simulink model "ESSSimulation_NCR"  (R2025a)
settings: Solver=VariableStepAuto  StartTime=0.0  StopTime=1800  RelTol=1e-3
undefined symbols (not defined in the file or in its folder): battery_builder_rtmsupport, gcbh
libraries: NCR18650BD_98S45P_Library_lib x14, fl_lib x4, nesl_utility x4, simulink x1, SignalEditorBlockLib x1
(part 1 of 2)
settings Model: Creator=saarv  LastModifiedBy=saarv

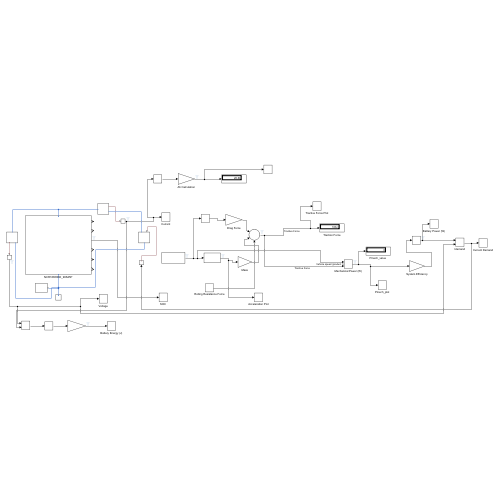
[thumbnail: Simulink's stored preview of the top-level diagram]
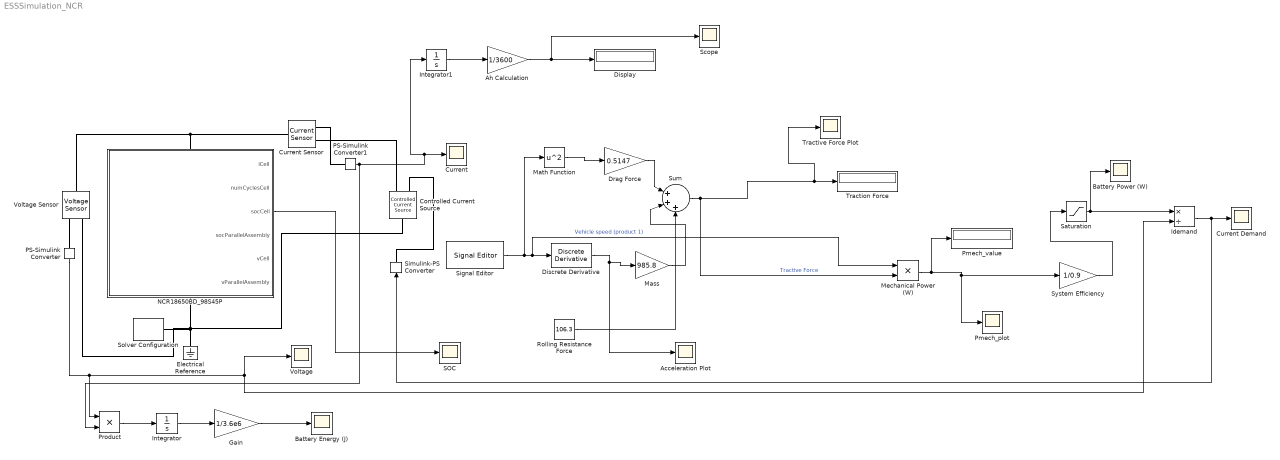
== system ESSSimulation_NCR ==
  Acceleration Plot : Scope
      settings: ActiveDisplayYMinimum=-1  ActiveDisplayYMaximum=1  DataLoggingVariableName=ScopeData3
  Ah Calculation : Gain  Gain=1/3600
  Battery Energy (J) : Scope
      settings: ActiveDisplayYMinimum=-1  ActiveDisplayYMaximum=1  DataLoggingVariableName=ScopeData8
  Battery Power (W) : Scope
      settings: ActiveDisplayYMinimum=-1660.4480803591648  ActiveDisplayYMaximum=14944.032723232487  DataLoggingVariableName=ScopeData6
  Controlled Current Source : fl_lib/Electrical/Electrical Sources/Controlled Current Source
  Current : Scope
      settings: ActiveDisplayYMinimum=-4.1863215438734489  ActiveDisplayYMaximum=37.676893894861045
  Current Demand : Scope
      settings: ActiveDisplayYMinimum=-4.1462072619256087  ActiveDisplayYMaximum=37.315865357330487  DataLoggingVariableName=ScopeData7
  Current Sensor : fl_lib/Electrical/Electrical Sensors/Current Sensor
  Discrete Derivative : simulink/Discrete/Discrete Derivative  gainval=1.0  ICPrevScaledInput=0.0  OutMin=[]  OutMax=[]  OutDataType=fixdt(1, 16)  OutScaling=2^-10  DoSatur=off
  Display : Display
  Drag Force : Gain  Gain=0.5147
  Electrical Reference : fl_lib/Electrical/Electrical Elements/Electrical Reference
  Gain : Gain  Gain=1/3.6e6
  Idemand : Product  Inputs=*/
  Integrator : Integrator
  Integrator1 : Integrator
  Mass : Gain  Gain=985.8
  Math Function : Math  Operator=square
  Mechanical Power (W) : Product
  NCR18650BD_98S45P : Subsystem  LoadFcn=battery_builder_rtmsupport('loadfcn',gcbh);
      settings: CopyFcn=battery_builder_rtmsupport('copyfcn',gcbh);  PreCopyFcn=battery_builder_rtmsupport('precopyfcn',gcbh);  PreDeleteFcn=battery_builder_rtmsupport('predeletefcn',gcbh);  PortSchema="{\"entries\":[{\"content\":{\"sides\":[{\"content\":{\"connectorIds\":[\"LConn1\"]},\"type\":\"ConnectorPlacement.EquallySpacedRectSide\",\"uuid\":\"9e7041d5-d3d9-4996-bd95-b169094aaa75\"},{\"content\":{\"connectorIds\":[\"RConn1\"],\"side\":\"RIGHT\"},\"type\":\"ConnectorPlacement.EquallySpacedRectSide\",\"uuid\":\"1a9d726b-e110-445d-9094-f9af8985733a\"},{\"content\":{\"side\":\"TOP\"},\"type\":\"ConnectorPlacement.EquallySpacedRectSide\",\"uuid\":\"c9094138-05f6-46bf-9d7c-2f9307e18b10\"},{\"content\":{\"connectorIds\":[\"Out1\",\"Out2\",\"Out3\",\"Out4\",\"Out5\",\"Out6\"],\"side\":\"BOTTOM\"},\"type\":\"ConnectorPlacement.EquallySpacedRectSide\",\"uuid\":\"12959d5d-2702-4b18-986c-5ba3b231edc9\"}]},\"type\":\"ConnectorPlacement.EquallySpacedConnector\",\"uuid\":\"b4792a63-91de-4aa8-9329-1ac229a09e41\"}],\"packageUris\":[\"http://schema.mathworks.com/mf0/Connector/R2020b\"],\"version\":\"1.0\"}"
      mask Display: image('$imagefile')
  PS-Simulink Converter : nesl_utility/PS-Simulink Converter  PhysicalDomain=network_engine_domain  SubClassName=ps_output  LeftPortType=input  RightPortType=output  PseudoPeriodic=off  Frequencies=[]  VectorFormat=inherit  Unit=inherit  AffineConversion=off
  PS-Simulink Converter1 : nesl_utility/PS-Simulink Converter  PhysicalDomain=network_engine_domain  SubClassName=ps_output  LeftPortType=input  RightPortType=output  PseudoPeriodic=off  Frequencies=[]  VectorFormat=inherit  Unit=inherit  AffineConversion=off
  Pmech_plot : Scope
      settings: ActiveDisplayYMinimum=-4360.824190842518  ActiveDisplayYMaximum=13768.120664078046  DataLoggingVariableName=ScopeData5
  "Pmech_value " : Display
  Product : Product
  Rolling Resistance Force : Constant  Value=106.3
  SOC : Scope
      settings: ActiveDisplayYMinimum=0.95619971788129954  ActiveDisplayYMaximum=1.0048666980131891  DataLoggingVariableName=ScopeData2
  Saturation : Saturate  UpperLimit=inf  LowerLimit=0
  Scope : Scope
      settings: ActiveDisplayYMinimum=-1  ActiveDisplayYMaximum=1  DataLoggingVariableName=ScopeData9
  Signal Editor : SignalEditorBlockLib/Signal Editor  FileName=EV_DriveProfiles.mat  ActiveScenario=SportProfile  ActiveSignal=VehicleSpeed  IsBus=off  OutputBusObjectStr=Bus: BusObject  SampleTime=10  ZeroCross=off  OutputAfterFinalValue=Setting to zero  Unit=m/s  PreserveSignalName=on  ApplySigPropsToAllScenarios=on  ApplySigPropsToAllSignals=off  SignalPropertySource=Dialog parameters
  Simulink-PS Converter : nesl_utility/Simulink-PS Converter  PhysicalDomain=network_engine_domain  SubClassName=ps_input  LeftPortType=input  RightPortType=output  PseudoPeriodic=off  Frequencies=[]  NoiseDistribution=none  NoiseParameters=[]  Unit=A  AffineConversion=off  FilteringAndDerivatives=provide  SimscapeFilterOrder=1  InputFilterTimeConstant=0.001  UdotUserProvided=0
  Solver Configuration : nesl_utility/Solver Configuration  PhysicalDomain=network_engine_domain  SubClassName=solver  LeftPortType=input  RightPortType=generic  Tones=[]  Harmonics=[]  SimulateNoise=off  Profile=off  UseLocalSampling=off  EnableSwitchedLinearOptims=on  FrequencyDomain=off  UseCCode=off  RelTol=0.001  AbsTol=0.001  MinStep=1e-09  ToWorkspace=off  RevertToSquareIcSolve=off  NumHomotopyIterations=100  PhasorMode=off  PhasorModeNumHarmonics=1  ConsistencySolver=NEWTON_XTOL_AFTER_FTOL  IndexReductionMethod=DerivativeReplacement  DoDC=off  ResidualTolerance=1e-09  ConsistencyTolSource=GLOBAL  ConsistencyAbsTol=0.001  ConsistencyRelTol=0.001  ConsistencyTolFactor=0.001  UseLocalSolver=off  LocalSolverChoice=NE_BACKWARD_EULER_ADVANCER  ResolveIndetEquations=on  FunctionEvalNumThread=1  LocalSolverSampleTime=0.001  DoFixedCost=off  MaxNonlinIter=3  MaxModeIter=2  ComputeImpulses=off  ImpulseIterations=2  LinearAlgebra=auto  LinearAlgebraNumThread=0  EquationFormulation=NE_TIME_EF  DelaysMemoryBudget=1024  AutomaticFiltering=on  FilteringTimeConstant=0.001  PartitionStorageMethod=AS_NEEDED  PartitionMemoryBudget=1024  PartitionMethod=ROBUST  MultibodyUseLocalSolver=off  MultibodyLocalSolverChoice=ODE1  MultibodyLocalSolverSampleTime=0.001
  Sum : Sum  Inputs=|+++
  System Efficiency : Gain  Gain=1/0.9
  Traction Force : Display
  Tractive Force Plot : Scope
      settings: ActiveDisplayYMinimum=-1  ActiveDisplayYMaximum=1  DataLoggingVariableName=ScopeData4
  Voltage : Scope
      settings: ActiveDisplayYMinimum=395.47317775463534  ActiveDisplayYMaximum=402.99624691615156
  Voltage Sensor : fl_lib/Electrical/Electrical Sensors/Voltage Sensor
  wires:
  PS-Simulink Converter/1 -> Product/1, Idemand/2, Voltage/1
  PS-Simulink Converter1/1 -> Product/2, Integrator1/1, Current/1
  Signal Editor/1 -> Math Function/1, Discrete Derivative/1, Mechanical Power (W)/1  "Vehicle speed (product 1)"
  Math Function/1 -> Drag Force/1
  Discrete Derivative/1 -> Acceleration Plot/1, Mass/1
  Drag Force/1 -> Sum/1
  Mass/1 -> Sum/2
  Rolling Resistance Force/1 -> Sum/3
  Sum/1 -> Mechanical Power (W)/2, Tractive Force Plot/1, Traction Force/1  "Tractive Force"
  Mechanical Power (W)/1 -> System Efficiency/1, Pmech_plot/1, "Pmech_value "/1
  System Efficiency/1 -> Saturation/1
  Saturation/1 -> Idemand/1, Battery Power (W)/1
  Idemand/1 -> Simulink-PS Converter/1, Current Demand/1
  Product/1 -> Integrator/1
  Integrator/1 -> Gain/1
  Gain/1 -> Battery Energy (J)/1
  Integrator1/1 -> Ah Calculation/1
  Ah Calculation/1 -> Scope/1, Display/1
  NCR18650BD_98S45P/3(socCell) -> SOC/1
  connections:
  Voltage Sensor/LConn1 -- NCR18650BD_98S45P/LConn1 -- Current Sensor/LConn1
  Electrical Reference/LConn1 -- NCR18650BD_98S45P/RConn1 -- Controlled Current Source/LConn1 -- Voltage Sensor/RConn2 -- Solver Configuration/RConn1
  Simulink-PS Converter/RConn1 -- Controlled Current Source/RConn1
  Voltage Sensor/RConn1 -- PS-Simulink Converter/LConn1
  Current Sensor/RConn1 -- PS-Simulink Converter1/LConn1
  Controlled Current Source/RConn2 -- Current Sensor/RConn2

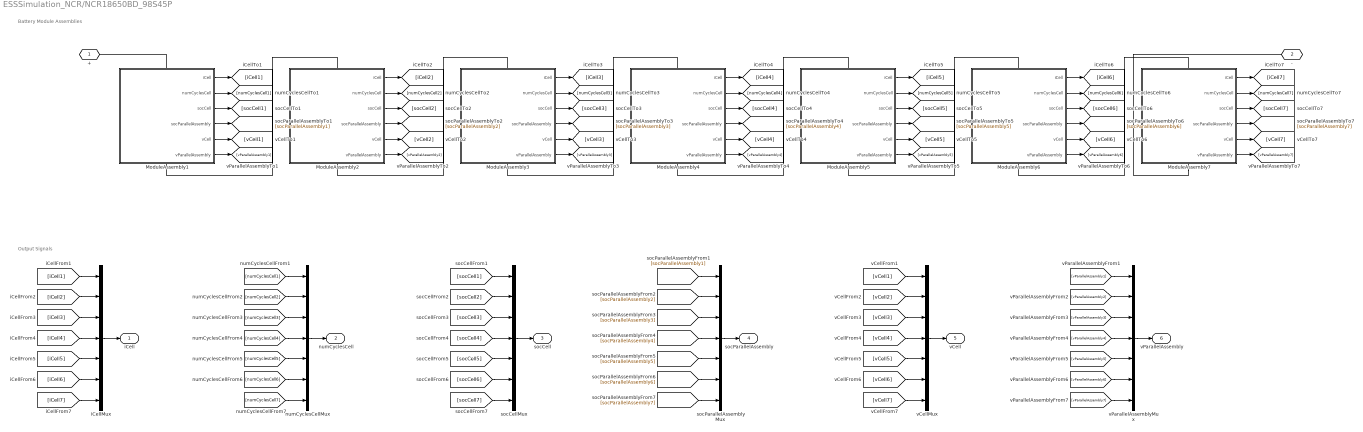
== system ESSSimulation_NCR/NCR18650BD_98S45P ==
  note: Output Signals
  note: Battery Module Assemblies
  ModuleAssembly1 : Subsystem  LoadFcn=battery_builder_rtmsupport('loadfcn',gcbh);
      settings: CopyFcn=battery_builder_rtmsupport('copyfcn',gcbh);  PreCopyFcn=battery_builder_rtmsupport('precopyfcn',gcbh);  PreDeleteFcn=battery_builder_rtmsupport('predeletefcn',gcbh);  PortSchema="{\"entries\":[{\"content\":{\"sides\":[{\"content\":{\"connectorIds\":[\"LConn1\"]},\"type\":\"ConnectorPlacement.EquallySpacedRectSide\",\"uuid\":\"9e7041d5-d3d9-4996-bd95-b169094aaa75\"},{\"content\":{\"connectorIds\":[\"RConn1\"],\"side\":\"RIGHT\"},\"type\":\"ConnectorPlacement.EquallySpacedRectSide\",\"uuid\":\"1a9d726b-e110-445d-9094-f9af8985733a\"},{\"content\":{\"side\":\"TOP\"},\"type\":\"ConnectorPlacement.EquallySpacedRectSide\",\"uuid\":\"c9094138-05f6-46bf-9d7c-2f9307e18b10\"},{\"content\":{\"connectorIds\":[\"Out1\",\"Out2\",\"Out3\",\"Out4\",\"Out5\",\"Out6\"],\"side\":\"BOTTOM\"},\"type\":\"ConnectorPlacement.EquallySpacedRectSide\",\"uuid\":\"a73cbc57-fefd-438e-a02a-7299c4782ae8\"}]},\"type\":\"ConnectorPlacement.EquallySpacedConnector\",\"uuid\":\"b4792a63-91de-4aa8-9329-1ac229a09e41\"}],\"packageUris\":[\"http://schema.mathworks.com/mf0/Connector/R2020b\"],\"version\":\"1.0\"}"
      mask Display: image('$imagefile')
  ModuleAssembly2 : Subsystem  LoadFcn=battery_builder_rtmsupport('loadfcn',gcbh);
      settings: CopyFcn=battery_builder_rtmsupport('copyfcn',gcbh);  PreCopyFcn=battery_builder_rtmsupport('precopyfcn',gcbh);  PreDeleteFcn=battery_builder_rtmsupport('predeletefcn',gcbh);  PortSchema="{\"entries\":[{\"content\":{\"sides\":[{\"content\":{\"connectorIds\":[\"LConn1\"]},\"type\":\"ConnectorPlacement.EquallySpacedRectSide\",\"uuid\":\"9e7041d5-d3d9-4996-bd95-b169094aaa75\"},{\"content\":{\"connectorIds\":[\"RConn1\"],\"side\":\"RIGHT\"},\"type\":\"ConnectorPlacement.EquallySpacedRectSide\",\"uuid\":\"1a9d726b-e110-445d-9094-f9af8985733a\"},{\"content\":{\"side\":\"TOP\"},\"type\":\"ConnectorPlacement.EquallySpacedRectSide\",\"uuid\":\"c9094138-05f6-46bf-9d7c-2f9307e18b10\"},{\"content\":{\"connectorIds\":[\"Out1\",\"Out2\",\"Out3\",\"Out4\",\"Out5\",\"Out6\"],\"side\":\"BOTTOM\"},\"type\":\"ConnectorPlacement.EquallySpacedRectSide\",\"uuid\":\"a73cbc57-fefd-438e-a02a-7299c4782ae8\"}]},\"type\":\"ConnectorPlacement.EquallySpacedConnector\",\"uuid\":\"b4792a63-91de-4aa8-9329-1ac229a09e41\"}],\"packageUris\":[\"http://schema.mathworks.com/mf0/Connector/R2020b\"],\"version\":\"1.0\"}"
      mask Display: image('moduleAssembly_1.JPG');
  ModuleAssembly3 : Subsystem  LoadFcn=battery_builder_rtmsupport('loadfcn',gcbh);
      settings: CopyFcn=battery_builder_rtmsupport('copyfcn',gcbh);  PreCopyFcn=battery_builder_rtmsupport('precopyfcn',gcbh);  PreDeleteFcn=battery_builder_rtmsupport('predeletefcn',gcbh);  PortSchema="{\"entries\":[{\"content\":{\"sides\":[{\"content\":{\"connectorIds\":[\"LConn1\"]},\"type\":\"ConnectorPlacement.EquallySpacedRectSide\",\"uuid\":\"9e7041d5-d3d9-4996-bd95-b169094aaa75\"},{\"content\":{\"connectorIds\":[\"RConn1\"],\"side\":\"RIGHT\"},\"type\":\"ConnectorPlacement.EquallySpacedRectSide\",\"uuid\":\"1a9d726b-e110-445d-9094-f9af8985733a\"},{\"content\":{\"side\":\"TOP\"},\"type\":\"ConnectorPlacement.EquallySpacedRectSide\",\"uuid\":\"c9094138-05f6-46bf-9d7c-2f9307e18b10\"},{\"content\":{\"connectorIds\":[\"Out1\",\"Out2\",\"Out3\",\"Out4\",\"Out5\",\"Out6\"],\"side\":\"BOTTOM\"},\"type\":\"ConnectorPlacement.EquallySpacedRectSide\",\"uuid\":\"a73cbc57-fefd-438e-a02a-7299c4782ae8\"}]},\"type\":\"ConnectorPlacement.EquallySpacedConnector\",\"uuid\":\"b4792a63-91de-4aa8-9329-1ac229a09e41\"}],\"packageUris\":[\"http://schema.mathworks.com/mf0/Connector/R2020b\"],\"version\":\"1.0\"}"
      mask Display: image('moduleAssembly_2.JPG');
  ModuleAssembly4 : Subsystem  LoadFcn=battery_builder_rtmsupport('loadfcn',gcbh);
      settings: CopyFcn=battery_builder_rtmsupport('copyfcn',gcbh);  PreCopyFcn=battery_builder_rtmsupport('precopyfcn',gcbh);  PreDeleteFcn=battery_builder_rtmsupport('predeletefcn',gcbh);  PortSchema="{\"entries\":[{\"content\":{\"sides\":[{\"content\":{\"connectorIds\":[\"LConn1\"]},\"type\":\"ConnectorPlacement.EquallySpacedRectSide\",\"uuid\":\"9e7041d5-d3d9-4996-bd95-b169094aaa75\"},{\"content\":{\"connectorIds\":[\"RConn1\"],\"side\":\"RIGHT\"},\"type\":\"ConnectorPlacement.EquallySpacedRectSide\",\"uuid\":\"1a9d726b-e110-445d-9094-f9af8985733a\"},{\"content\":{\"side\":\"TOP\"},\"type\":\"ConnectorPlacement.EquallySpacedRectSide\",\"uuid\":\"c9094138-05f6-46bf-9d7c-2f9307e18b10\"},{\"content\":{\"connectorIds\":[\"Out1\",\"Out2\",\"Out3\",\"Out4\",\"Out5\",\"Out6\"],\"side\":\"BOTTOM\"},\"type\":\"ConnectorPlacement.EquallySpacedRectSide\",\"uuid\":\"a73cbc57-fefd-438e-a02a-7299c4782ae8\"}]},\"type\":\"ConnectorPlacement.EquallySpacedConnector\",\"uuid\":\"b4792a63-91de-4aa8-9329-1ac229a09e41\"}],\"packageUris\":[\"http://schema.mathworks.com/mf0/Connector/R2020b\"],\"version\":\"1.0\"}"
      mask Display: image('moduleAssembly_3.JPG');
  ModuleAssembly5 : Subsystem  LoadFcn=battery_builder_rtmsupport('loadfcn',gcbh);
      settings: CopyFcn=battery_builder_rtmsupport('copyfcn',gcbh);  PreCopyFcn=battery_builder_rtmsupport('precopyfcn',gcbh);  PreDeleteFcn=battery_builder_rtmsupport('predeletefcn',gcbh);  PortSchema="{\"entries\":[{\"content\":{\"sides\":[{\"content\":{\"connectorIds\":[\"LConn1\"]},\"type\":\"ConnectorPlacement.EquallySpacedRectSide\",\"uuid\":\"9e7041d5-d3d9-4996-bd95-b169094aaa75\"},{\"content\":{\"connectorIds\":[\"RConn1\"],\"side\":\"RIGHT\"},\"type\":\"ConnectorPlacement.EquallySpacedRectSide\",\"uuid\":\"1a9d726b-e110-445d-9094-f9af8985733a\"},{\"content\":{\"side\":\"TOP\"},\"type\":\"ConnectorPlacement.EquallySpacedRectSide\",\"uuid\":\"c9094138-05f6-46bf-9d7c-2f9307e18b10\"},{\"content\":{\"connectorIds\":[\"Out1\",\"Out2\",\"Out3\",\"Out4\",\"Out5\",\"Out6\"],\"side\":\"BOTTOM\"},\"type\":\"ConnectorPlacement.EquallySpacedRectSide\",\"uuid\":\"a73cbc57-fefd-438e-a02a-7299c4782ae8\"}]},\"type\":\"ConnectorPlacement.EquallySpacedConnector\",\"uuid\":\"b4792a63-91de-4aa8-9329-1ac229a09e41\"}],\"packageUris\":[\"http://schema.mathworks.com/mf0/Connector/R2020b\"],\"version\":\"1.0\"}"
      mask Display: image('moduleAssembly_4.JPG');
  ModuleAssembly6 : Subsystem  LoadFcn=battery_builder_rtmsupport('loadfcn',gcbh);
      settings: CopyFcn=battery_builder_rtmsupport('copyfcn',gcbh);  PreCopyFcn=battery_builder_rtmsupport('precopyfcn',gcbh);  PreDeleteFcn=battery_builder_rtmsupport('predeletefcn',gcbh);  PortSchema="{\"entries\":[{\"content\":{\"sides\":[{\"content\":{\"connectorIds\":[\"LConn1\"]},\"type\":\"ConnectorPlacement.EquallySpacedRectSide\",\"uuid\":\"9e7041d5-d3d9-4996-bd95-b169094aaa75\"},{\"content\":{\"connectorIds\":[\"RConn1\"],\"side\":\"RIGHT\"},\"type\":\"ConnectorPlacement.EquallySpacedRectSide\",\"uuid\":\"1a9d726b-e110-445d-9094-f9af8985733a\"},{\"content\":{\"side\":\"TOP\"},\"type\":\"ConnectorPlacement.EquallySpacedRectSide\",\"uuid\":\"c9094138-05f6-46bf-9d7c-2f9307e18b10\"},{\"content\":{\"connectorIds\":[\"Out1\",\"Out2\",\"Out3\",\"Out4\",\"Out5\",\"Out6\"],\"side\":\"BOTTOM\"},\"type\":\"ConnectorPlacement.EquallySpacedRectSide\",\"uuid\":\"a73cbc57-fefd-438e-a02a-7299c4782ae8\"}]},\"type\":\"ConnectorPlacement.EquallySpacedConnector\",\"uuid\":\"b4792a63-91de-4aa8-9329-1ac229a09e41\"}],\"packageUris\":[\"http://schema.mathworks.com/mf0/Connector/R2020b\"],\"version\":\"1.0\"}"
      mask Display: image('moduleAssembly_5.JPG');
  ModuleAssembly7 : Subsystem  LoadFcn=battery_builder_rtmsupport('loadfcn',gcbh);
      settings: CopyFcn=battery_builder_rtmsupport('copyfcn',gcbh);  PreCopyFcn=battery_builder_rtmsupport('precopyfcn',gcbh);  PreDeleteFcn=battery_builder_rtmsupport('predeletefcn',gcbh);  PortSchema="{\"entries\":[{\"content\":{\"sides\":[{\"content\":{\"connectorIds\":[\"LConn1\"]},\"type\":\"ConnectorPlacement.EquallySpacedRectSide\",\"uuid\":\"9e7041d5-d3d9-4996-bd95-b169094aaa75\"},{\"content\":{\"connectorIds\":[\"RConn1\"],\"side\":\"RIGHT\"},\"type\":\"ConnectorPlacement.EquallySpacedRectSide\",\"uuid\":\"1a9d726b-e110-445d-9094-f9af8985733a\"},{\"content\":{\"side\":\"TOP\"},\"type\":\"ConnectorPlacement.EquallySpacedRectSide\",\"uuid\":\"c9094138-05f6-46bf-9d7c-2f9307e18b10\"},{\"content\":{\"connectorIds\":[\"Out1\",\"Out2\",\"Out3\",\"Out4\",\"Out5\",\"Out6\"],\"side\":\"BOTTOM\"},\"type\":\"ConnectorPlacement.EquallySpacedRectSide\",\"uuid\":\"a73cbc57-fefd-438e-a02a-7299c4782ae8\"}]},\"type\":\"ConnectorPlacement.EquallySpacedConnector\",\"uuid\":\"b4792a63-91de-4aa8-9329-1ac229a09e41\"}],\"packageUris\":[\"http://schema.mathworks.com/mf0/Connector/R2020b\"],\"version\":\"1.0\"}"
      mask Display: image('moduleAssembly_6.JPG');
  iCellMux : Mux  Inputs=7
  numCyclesCellMux : Mux  Inputs=7
  socCellMux : Mux  Inputs=7
  socParallelAssemblyMux : Mux  Inputs=7
  vCellMux : Mux  Inputs=7
  vParallelAssemblyMux : Mux  Inputs=7
  + : PMIOPort  Side=Left
  - : PMIOPort  Port=2  Side=Right
  iCell : Outport
  numCyclesCell : Outport  Port=2
  socCell : Outport  Port=3
  socParallelAssembly : Outport  Port=4
  vCell : Outport  Port=5
  vParallelAssembly : Outport  Port=6
  wires:
  [vParallelAssembly7] -> vParallelAssemblyMux/7
  ModuleAssembly7/6(vParallelAssembly) -> [vParallelAssembly7]
  [vCell7] -> vCellMux/7
  ModuleAssembly7/5(vCell) -> [vCell7]
  [socParallelAssembly7] -> socParallelAssemblyMux/7
  ModuleAssembly7/4(socParallelAssembly) -> [socParallelAssembly7]
  [socCell7] -> socCellMux/7
  ModuleAssembly7/3(socCell) -> [socCell7]
  [numCyclesCell7] -> numCyclesCellMux/7
  ModuleAssembly7/2(numCyclesCell) -> [numCyclesCell7]
  [iCell7] -> iCellMux/7
  ModuleAssembly7/1(iCell) -> [iCell7]
  [vParallelAssembly6] -> vParallelAssemblyMux/6
  ModuleAssembly6/6(vParallelAssembly) -> [vParallelAssembly6]
  [vCell6] -> vCellMux/6
  ModuleAssembly6/5(vCell) -> [vCell6]
  [socParallelAssembly6] -> socParallelAssemblyMux/6
  ModuleAssembly6/4(socParallelAssembly) -> [socParallelAssembly6]
  [socCell6] -> socCellMux/6
  ModuleAssembly6/3(socCell) -> [socCell6]
  [numCyclesCell6] -> numCyclesCellMux/6
  ModuleAssembly6/2(numCyclesCell) -> [numCyclesCell6]
  [iCell6] -> iCellMux/6
  ModuleAssembly6/1(iCell) -> [iCell6]
  [vParallelAssembly5] -> vParallelAssemblyMux/5
  ModuleAssembly5/6(vParallelAssembly) -> [vParallelAssembly5]
  [vCell5] -> vCellMux/5
  ModuleAssembly5/5(vCell) -> [vCell5]
  [socParallelAssembly5] -> socParallelAssemblyMux/5
  ModuleAssembly5/4(socParallelAssembly) -> [socParallelAssembly5]
  [socCell5] -> socCellMux/5
  ModuleAssembly5/3(socCell) -> [socCell5]
  [numCyclesCell5] -> numCyclesCellMux/5
  ModuleAssembly5/2(numCyclesCell) -> [numCyclesCell5]
  [iCell5] -> iCellMux/5
  ModuleAssembly5/1(iCell) -> [iCell5]
  [vParallelAssembly4] -> vParallelAssemblyMux/4
  ModuleAssembly4/6(vParallelAssembly) -> [vParallelAssembly4]
  [vCell4] -> vCellMux/4
  ModuleAssembly4/5(vCell) -> [vCell4]
  [socParallelAssembly4] -> socParallelAssemblyMux/4
  ModuleAssembly4/4(socParallelAssembly) -> [socParallelAssembly4]
  [socCell4] -> socCellMux/4
  ModuleAssembly4/3(socCell) -> [socCell4]
  [numCyclesCell4] -> numCyclesCellMux/4
  ModuleAssembly4/2(numCyclesCell) -> [numCyclesCell4]
  [iCell4] -> iCellMux/4
  ModuleAssembly4/1(iCell) -> [iCell4]
  [vParallelAssembly3] -> vParallelAssemblyMux/3
  ModuleAssembly3/6(vParallelAssembly) -> [vParallelAssembly3]
  [vCell3] -> vCellMux/3
  ModuleAssembly3/5(vCell) -> [vCell3]
  [socParallelAssembly3] -> socParallelAssemblyMux/3
  ModuleAssembly3/4(socParallelAssembly) -> [socParallelAssembly3]
  [socCell3] -> socCellMux/3
  ModuleAssembly3/3(socCell) -> [socCell3]
  [numCyclesCell3] -> numCyclesCellMux/3
  ModuleAssembly3/2(numCyclesCell) -> [numCyclesCell3]
  [iCell3] -> iCellMux/3
  ModuleAssembly3/1(iCell) -> [iCell3]
  [vParallelAssembly2] -> vParallelAssemblyMux/2
  ModuleAssembly2/6(vParallelAssembly) -> [vParallelAssembly2]
  [vCell2] -> vCellMux/2
  ModuleAssembly2/5(vCell) -> [vCell2]
  [socParallelAssembly2] -> socParallelAssemblyMux/2
  ModuleAssembly2/4(socParallelAssembly) -> [socParallelAssembly2]
  [socCell2] -> socCellMux/2
  ModuleAssembly2/3(socCell) -> [socCell2]
  [numCyclesCell2] -> numCyclesCellMux/2
  ModuleAssembly2/2(numCyclesCell) -> [numCyclesCell2]
  [iCell2] -> iCellMux/2
  ModuleAssembly2/1(iCell) -> [iCell2]
  [vParallelAssembly1] -> vParallelAssemblyMux/1
  vParallelAssemblyMux/1 -> vParallelAssembly/1
  ModuleAssembly1/6(vParallelAssembly) -> [vParallelAssembly1]
  [vCell1] -> vCellMux/1
  vCellMux/1 -> vCell/1
  ModuleAssembly1/5(vCell) -> [vCell1]
  [socParallelAssembly1] -> socParallelAssemblyMux/1
  socParallelAssemblyMux/1 -> socParallelAssembly/1
  ModuleAssembly1/4(socParallelAssembly) -> [socParallelAssembly1]
  [socCell1] -> socCellMux/1
  socCellMux/1 -> socCell/1
  ModuleAssembly1/3(socCell) -> [socCell1]
  [numCyclesCell1] -> numCyclesCellMux/1
  numCyclesCellMux/1 -> numCyclesCell/1
  ModuleAssembly1/2(numCyclesCell) -> [numCyclesCell1]
  [iCell1] -> iCellMux/1
  iCellMux/1 -> iCell/1
  ModuleAssembly1/1(iCell) -> [iCell1]
  connections:
  ModuleAssembly7/RConn1 -- -/RConn1
  ModuleAssembly1/LConn1 -- +/RConn1
  ModuleAssembly7/LConn1 -- ModuleAssembly6/RConn1
  ModuleAssembly6/LConn1 -- ModuleAssembly5/RConn1
  ModuleAssembly5/LConn1 -- ModuleAssembly4/RConn1
  ModuleAssembly4/LConn1 -- ModuleAssembly3/RConn1
  ModuleAssembly3/LConn1 -- ModuleAssembly2/RConn1
  ModuleAssembly2/LConn1 -- ModuleAssembly1/RConn1

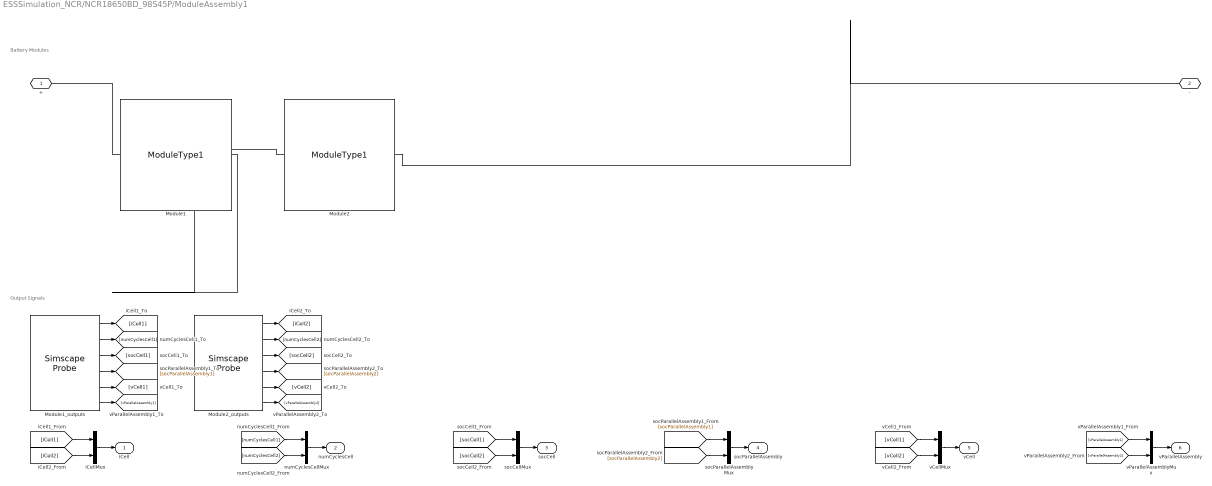
== system ESSSimulation_NCR/NCR18650BD_98S45P/ModuleAssembly1 ==
  note: Battery Modules
  note: Output Signals
  Module1 : NCR18650BD_98S45P_Library_lib/Modules/ModuleType1  SOC_vecCell=[0 0.01 0.02 0.03 0.04 0.05 0.06 0.07 0.08 0.09 0.1 0.11 0.12 0.13 0.14 0.15 0.16 0.17 0.18 0.19 0.2 0.21 0.22 0.23 0.24 0.25 0.26 0.27 0.28 0.29 0.3 0.31 0.32 0.33 0.34 0.35 0.36 0.37 0.38 0.39 0.4 0.41 0.42 0.43 0.44 0.45 0.46 0.47 0.48 0.49 0.5 0.51 0.52 0.53 0.54 0.55 0.56 0.57 0.58 0.59 0.6 0.61 0.62 0.63 0.64 0.65 0.66 0.67 0.68 0.69 0.7 0.71 0.72 0.73 0.74 0.75 0.76 0.77 0.78 0.79 0.8 0.81 0.82 0.83 0.84 0.85 0.86 0.87 0.88 0.89 0.9 0.91 0.92 0.93 0.94 0.95 0.96 0.97 0.98 0.99 1]  V0_vecCell=[2.90003 2.94341 2.98679 3.04987 3.09433 3.12791 3.16031 3.20369 3.23862 3.26689 3.29115 3.31383 3.33202 3.35112 3.36833 3.38413 3.39973 3.41137 3.42149 3.43136 3.44073 3.45027 3.46068 3.47113 3.47814 3.48494 3.49199 3.49905 3.50562 3.51187 3.51861 3.52535 3.53209 3.53818 3.54353 3.54849 3.55353 3.55855 3.56357 3.56831 3.57308 3.57787 3.58264 3.58755 3.5925 3.5985 3.60496 3.61149 3.61805 3.6246 3.63116 3.63855 3.64609 3.65336 3.66064 3.66791 3.67613 3.68522 3.69443 3.70367 3.713 3.72241 3.73154 3.74037 3.7492 3.75786 3.76617 3.77556 3.78485 3.79413 3.8034 3.81149 3.81977 3.82804 3.83631 3.84472 3.85317 3.86155 3.86993 3.87831 3.88686 3.89534 3.90461 3.91454 3.92565 3.93721 3.94924 3.96155 3.97383 3.98598 3.99856 4.01117 4.02361 4.03609 4.04694 4.05695 4.06641 4.07551 4.08514 4.09447 4.10453] V  V_rangeCell=[2.25 Inf] V  R0_vecCell=[0.1741 0.15823 0.14313 0.13285 0.12044 0.10641 0.09605 0.09162 0.08758 0.08349 0.08021 0.07738 0.07487 0.07338 0.07189 0.07117 0.0704 0.06898 0.06755 0.06631 0.06509 0.06388 0.06326 0.06281 0.06182 0.06095 0.06025 0.05955 0.05877 0.05807 0.05761 0.05714 0.05668 0.05611 0.05546 0.0549 0.05439 0.05388 0.05337 0.0528 0.05223 0.05165 0.05106 0.05046 0.04986 0.04945 0.04913 0.04883 0.04854 0.04826 0.04797 0.04782 0.04765 0.0473 0.04695 0.04661 0.04638 0.0463 0.04625 0.04621 0.04624 0.04628 0.04628 0.04623 0.04617 0.04599 0.04573 0.0457 0.04568 0.04565 0.04563 0.04535 0.0451 0.04486 0.04461 0.04446 0.04435 0.04423 0.04411 0.044 0.04372 0.04339 0.04323 0.0432 0.04344 0.04374 0.0441 0.04452 0.04494 0.0454 0.04594 0.0463 0.04649 0.04668 0.04629 0.04541 0.04438 0.04326 0.04154 0.03869 0.03326] Ohm  AHCell=3.153 hr*A  extrapolation_optionCell=simscape.enum.extrapolation.nearest  P=45  S=7  iCell_specify=off  iCell_priority=None  iCell=0 A  iCell_nominal_specify=off  iCell_nominal_value=1  iCell_nominal_unit=A  vCell_specify=off  vCell_priority=None  vCell=0 V  vCell_nominal_specify=off  vCell_nominal_value=1  vCell_nominal_unit=V  socCell_specify=off  socCell_priority=High  socCell=1  socCell_nominal_specify=off  socCell_nominal_value=1  socCell_nominal_unit=1  numCyclesCell_specify=off  numCyclesCell_priority=High  numCyclesCell=0  numCyclesCell_nominal_specify=off  numCyclesCell_nominal_value=1  numCyclesCell_nominal_unit=1  vParallelAssembly_specify=off  vParallelAssembly_priority=None  vParallelAssembly=repmat(0, 7, 1) V  vParallelAssembly_nominal_specify=off  vParallelAssembly_nominal_value=1  vParallelAssembly_nominal_unit=V  socParallelAssembly_specify=off  socParallelAssembly_priority=None  socParallelAssembly=repmat(1, 7, 1)  socParallelAssembly_nominal_specify=off  socParallelAssembly_nominal_value=1  socParallelAssembly_nominal_unit=1
      settings: InternalSimscapePortConfiguration="{\"Bottom\":[{\"id\":\"n\",\"label\":\"-\",\"type\":\"foundation.electrical.electrical\"}],\"Left\":[],\"Right\":[],\"Top\":[{\"id\":\"p\",\"label\":\"+\",\"type\":\"foundation.electrical.electrical\"}]}"
  Module1_outputs : SimscapeProbe  BoundBlock=600  Variables="{\"iCell\":{\"Probing\":\"ON\"},\"numCyclesCell\":{\"Probing\":\"ON\"},\"socCell\":{\"Probing\":\"ON\"},\"socParallelAssembly\":{\"Probing\":\"ON\"},\"vCell\":{\"Probing\":\"ON\"},\"vParallelAssembly\":{\"Probing\":\"ON\"}}"
  Module2 : NCR18650BD_98S45P_Library_lib/Modules/ModuleType1  SOC_vecCell=[0 0.01 0.02 0.03 0.04 0.05 0.06 0.07 0.08 0.09 0.1 0.11 0.12 0.13 0.14 0.15 0.16 0.17 0.18 0.19 0.2 0.21 0.22 0.23 0.24 0.25 0.26 0.27 0.28 0.29 0.3 0.31 0.32 0.33 0.34 0.35 0.36 0.37 0.38 0.39 0.4 0.41 0.42 0.43 0.44 0.45 0.46 0.47 0.48 0.49 0.5 0.51 0.52 0.53 0.54 0.55 0.56 0.57 0.58 0.59 0.6 0.61 0.62 0.63 0.64 0.65 0.66 0.67 0.68 0.69 0.7 0.71 0.72 0.73 0.74 0.75 0.76 0.77 0.78 0.79 0.8 0.81 0.82 0.83 0.84 0.85 0.86 0.87 0.88 0.89 0.9 0.91 0.92 0.93 0.94 0.95 0.96 0.97 0.98 0.99 1]  V0_vecCell=[2.90003 2.94341 2.98679 3.04987 3.09433 3.12791 3.16031 3.20369 3.23862 3.26689 3.29115 3.31383 3.33202 3.35112 3.36833 3.38413 3.39973 3.41137 3.42149 3.43136 3.44073 3.45027 3.46068 3.47113 3.47814 3.48494 3.49199 3.49905 3.50562 3.51187 3.51861 3.52535 3.53209 3.53818 3.54353 3.54849 3.55353 3.55855 3.56357 3.56831 3.57308 3.57787 3.58264 3.58755 3.5925 3.5985 3.60496 3.61149 3.61805 3.6246 3.63116 3.63855 3.64609 3.65336 3.66064 3.66791 3.67613 3.68522 3.69443 3.70367 3.713 3.72241 3.73154 3.74037 3.7492 3.75786 3.76617 3.77556 3.78485 3.79413 3.8034 3.81149 3.81977 3.82804 3.83631 3.84472 3.85317 3.86155 3.86993 3.87831 3.88686 3.89534 3.90461 3.91454 3.92565 3.93721 3.94924 3.96155 3.97383 3.98598 3.99856 4.01117 4.02361 4.03609 4.04694 4.05695 4.06641 4.07551 4.08514 4.09447 4.10453] V  V_rangeCell=[2.25 Inf] V  R0_vecCell=[0.1741 0.15823 0.14313 0.13285 0.12044 0.10641 0.09605 0.09162 0.08758 0.08349 0.08021 0.07738 0.07487 0.07338 0.07189 0.07117 0.0704 0.06898 0.06755 0.06631 0.06509 0.06388 0.06326 0.06281 0.06182 0.06095 0.06025 0.05955 0.05877 0.05807 0.05761 0.05714 0.05668 0.05611 0.05546 0.0549 0.05439 0.05388 0.05337 0.0528 0.05223 0.05165 0.05106 0.05046 0.04986 0.04945 0.04913 0.04883 0.04854 0.04826 0.04797 0.04782 0.04765 0.0473 0.04695 0.04661 0.04638 0.0463 0.04625 0.04621 0.04624 0.04628 0.04628 0.04623 0.04617 0.04599 0.04573 0.0457 0.04568 0.04565 0.04563 0.04535 0.0451 0.04486 0.04461 0.04446 0.04435 0.04423 0.04411 0.044 0.04372 0.04339 0.04323 0.0432 0.04344 0.04374 0.0441 0.04452 0.04494 0.0454 0.04594 0.0463 0.04649 0.04668 0.04629 0.04541 0.04438 0.04326 0.04154 0.03869 0.03326] Ohm  AHCell=3.153 hr*A  extrapolation_optionCell=simscape.enum.extrapolation.nearest  P=45  S=7  iCell_specify=off  iCell_priority=None  iCell=0 A  iCell_nominal_specify=off  iCell_nominal_value=1  iCell_nominal_unit=A  vCell_specify=off  vCell_priority=None  vCell=0 V  vCell_nominal_specify=off  vCell_nominal_value=1  vCell_nominal_unit=V  socCell_specify=off  socCell_priority=High  socCell=1  socCell_nominal_specify=off  socCell_nominal_value=1  socCell_nominal_unit=1  numCyclesCell_specify=off  numCyclesCell_priority=High  numCyclesCell=0  numCyclesCell_nominal_specify=off  numCyclesCell_nominal_value=1  numCyclesCell_nominal_unit=1  vParallelAssembly_specify=off  vParallelAssembly_priority=None  vParallelAssembly=repmat(0, 7, 1) V  vParallelAssembly_nominal_specify=off  vParallelAssembly_nominal_value=1  vParallelAssembly_nominal_unit=V  socParallelAssembly_specify=off  socParallelAssembly_priority=None  socParallelAssembly=repmat(1, 7, 1)  socParallelAssembly_nominal_specify=off  socParallelAssembly_nominal_value=1  socParallelAssembly_nominal_unit=1
      settings: InternalSimscapePortConfiguration="{\"Bottom\":[{\"id\":\"n\",\"label\":\"-\",\"type\":\"foundation.electrical.electrical\"}],\"Left\":[],\"Right\":[],\"Top\":[{\"id\":\"p\",\"label\":\"+\",\"type\":\"foundation.electrical.electrical\"}]}"
  Module2_outputs : SimscapeProbe  BoundBlock=602  Variables="{\"iCell\":{\"Probing\":\"ON\"},\"numCyclesCell\":{\"Probing\":\"ON\"},\"socCell\":{\"Probing\":\"ON\"},\"socParallelAssembly\":{\"Probing\":\"ON\"},\"vCell\":{\"Probing\":\"ON\"},\"vParallelAssembly\":{\"Probing\":\"ON\"}}"
  iCellMux : Mux  Inputs=2
  numCyclesCellMux : Mux  Inputs=2
  socCellMux : Mux  Inputs=2
  socParallelAssemblyMux : Mux  Inputs=2
  vCellMux : Mux  Inputs=2
  vParallelAssemblyMux : Mux  Inputs=2
  + : PMIOPort  Side=Left
  - : PMIOPort  Port=2  Side=Right
  iCell : Outport
  numCyclesCell : Outport  Port=2
  socCell : Outport  Port=3
  socParallelAssembly : Outport  Port=4
  vCell : Outport  Port=5
  vParallelAssembly : Outport  Port=6
  wires:
  Module1_outputs/1 -> [iCell1]
  iCellMux/1 -> iCell/1
  [iCell1] -> iCellMux/1
  Module1_outputs/2 -> [numCyclesCell1]
  numCyclesCellMux/1 -> numCyclesCell/1
  [numCyclesCell1] -> numCyclesCellMux/1
  Module1_outputs/3 -> [socCell1]
  socCellMux/1 -> socCell/1
  [socCell1] -> socCellMux/1
  Module1_outputs/4 -> [socParallelAssembly1]
  socParallelAssemblyMux/1 -> socParallelAssembly/1
  [socParallelAssembly1] -> socParallelAssemblyMux/1
  Module1_outputs/5 -> [vCell1]
  vCellMux/1 -> vCell/1
  [vCell1] -> vCellMux/1
  Module1_outputs/6 -> [vParallelAssembly1]
  vParallelAssemblyMux/1 -> vParallelAssembly/1
  [vParallelAssembly1] -> vParallelAssemblyMux/1
  Module2_outputs/1 -> [iCell2]
  [iCell2] -> iCellMux/2
  Module2_outputs/2 -> [numCyclesCell2]
  [numCyclesCell2] -> numCyclesCellMux/2
  Module2_outputs/3 -> [socCell2]
  [socCell2] -> socCellMux/2
  Module2_outputs/4 -> [socParallelAssembly2]
  [socParallelAssembly2] -> socParallelAssemblyMux/2
  Module2_outputs/5 -> [vCell2]
  [vCell2] -> vCellMux/2
  Module2_outputs/6 -> [vParallelAssembly2]
  [vParallelAssembly2] -> vParallelAssemblyMux/2
  connections:
  Module2/LConn1 -- Module1/RConn1
  Module1/LConn1 -- +/RConn1
  Module2/RConn1 -- -/RConn1

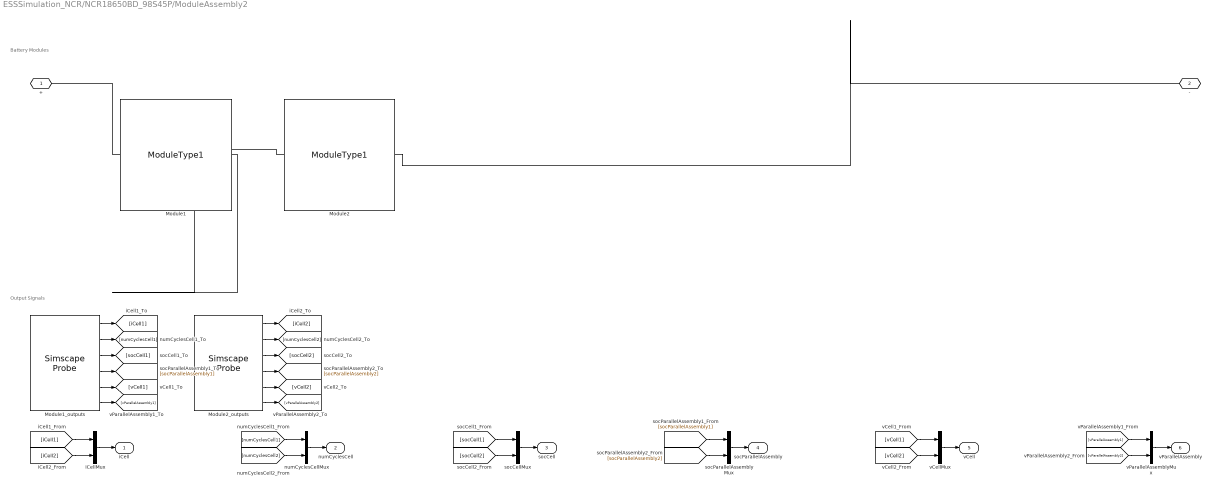
== system ESSSimulation_NCR/NCR18650BD_98S45P/ModuleAssembly2 ==
  note: Battery Modules
  note: Output Signals
  Module1 : NCR18650BD_98S45P_Library_lib/Modules/ModuleType1  SOC_vecCell=[0 0.01 0.02 0.03 0.04 0.05 0.06 0.07 0.08 0.09 0.1 0.11 0.12 0.13 0.14 0.15 0.16 0.17 0.18 0.19 0.2 0.21 0.22 0.23 0.24 0.25 0.26 0.27 0.28 0.29 0.3 0.31 0.32 0.33 0.34 0.35 0.36 0.37 0.38 0.39 0.4 0.41 0.42 0.43 0.44 0.45 0.46 0.47 0.48 0.49 0.5 0.51 0.52 0.53 0.54 0.55 0.56 0.57 0.58 0.59 0.6 0.61 0.62 0.63 0.64 0.65 0.66 0.67 0.68 0.69 0.7 0.71 0.72 0.73 0.74 0.75 0.76 0.77 0.78 0.79 0.8 0.81 0.82 0.83 0.84 0.85 0.86 0.87 0.88 0.89 0.9 0.91 0.92 0.93 0.94 0.95 0.96 0.97 0.98 0.99 1]  V0_vecCell=[2.90003 2.94341 2.98679 3.04987 3.09433 3.12791 3.16031 3.20369 3.23862 3.26689 3.29115 3.31383 3.33202 3.35112 3.36833 3.38413 3.39973 3.41137 3.42149 3.43136 3.44073 3.45027 3.46068 3.47113 3.47814 3.48494 3.49199 3.49905 3.50562 3.51187 3.51861 3.52535 3.53209 3.53818 3.54353 3.54849 3.55353 3.55855 3.56357 3.56831 3.57308 3.57787 3.58264 3.58755 3.5925 3.5985 3.60496 3.61149 3.61805 3.6246 3.63116 3.63855 3.64609 3.65336 3.66064 3.66791 3.67613 3.68522 3.69443 3.70367 3.713 3.72241 3.73154 3.74037 3.7492 3.75786 3.76617 3.77556 3.78485 3.79413 3.8034 3.81149 3.81977 3.82804 3.83631 3.84472 3.85317 3.86155 3.86993 3.87831 3.88686 3.89534 3.90461 3.91454 3.92565 3.93721 3.94924 3.96155 3.97383 3.98598 3.99856 4.01117 4.02361 4.03609 4.04694 4.05695 4.06641 4.07551 4.08514 4.09447 4.10453] V  V_rangeCell=[2.25 Inf] V  R0_vecCell=[0.1741 0.15823 0.14313 0.13285 0.12044 0.10641 0.09605 0.09162 0.08758 0.08349 0.08021 0.07738 0.07487 0.07338 0.07189 0.07117 0.0704 0.06898 0.06755 0.06631 0.06509 0.06388 0.06326 0.06281 0.06182 0.06095 0.06025 0.05955 0.05877 0.05807 0.05761 0.05714 0.05668 0.05611 0.05546 0.0549 0.05439 0.05388 0.05337 0.0528 0.05223 0.05165 0.05106 0.05046 0.04986 0.04945 0.04913 0.04883 0.04854 0.04826 0.04797 0.04782 0.04765 0.0473 0.04695 0.04661 0.04638 0.0463 0.04625 0.04621 0.04624 0.04628 0.04628 0.04623 0.04617 0.04599 0.04573 0.0457 0.04568 0.04565 0.04563 0.04535 0.0451 0.04486 0.04461 0.04446 0.04435 0.04423 0.04411 0.044 0.04372 0.04339 0.04323 0.0432 0.04344 0.04374 0.0441 0.04452 0.04494 0.0454 0.04594 0.0463 0.04649 0.04668 0.04629 0.04541 0.04438 0.04326 0.04154 0.03869 0.03326] Ohm  AHCell=3.153 hr*A  extrapolation_optionCell=simscape.enum.extrapolation.nearest  P=45  S=7  iCell_specify=off  iCell_priority=None  iCell=0 A  iCell_nominal_specify=off  iCell_nominal_value=1  iCell_nominal_unit=A  vCell_specify=off  vCell_priority=None  vCell=0 V  vCell_nominal_specify=off  vCell_nominal_value=1  vCell_nominal_unit=V  socCell_specify=off  socCell_priority=High  socCell=1  socCell_nominal_specify=off  socCell_nominal_value=1  socCell_nominal_unit=1  numCyclesCell_specify=off  numCyclesCell_priority=High  numCyclesCell=0  numCyclesCell_nominal_specify=off  numCyclesCell_nominal_value=1  numCyclesCell_nominal_unit=1  vParallelAssembly_specify=off  vParallelAssembly_priority=None  vParallelAssembly=repmat(0, 7, 1) V  vParallelAssembly_nominal_specify=off  vParallelAssembly_nominal_value=1  vParallelAssembly_nominal_unit=V  socParallelAssembly_specify=off  socParallelAssembly_priority=None  socParallelAssembly=repmat(1, 7, 1)  socParallelAssembly_nominal_specify=off  socParallelAssembly_nominal_value=1  socParallelAssembly_nominal_unit=1
      settings: InternalSimscapePortConfiguration="{\"Bottom\":[{\"id\":\"n\",\"label\":\"-\",\"type\":\"foundation.electrical.electrical\"}],\"Left\":[],\"Right\":[],\"Top\":[{\"id\":\"p\",\"label\":\"+\",\"type\":\"foundation.electrical.electrical\"}]}"
  Module1_outputs : SimscapeProbe  BoundBlock=645  Variables="{\"iCell\":{\"Probing\":\"ON\"},\"numCyclesCell\":{\"Probing\":\"ON\"},\"socCell\":{\"Probing\":\"ON\"},\"socParallelAssembly\":{\"Probing\":\"ON\"},\"vCell\":{\"Probing\":\"ON\"},\"vParallelAssembly\":{\"Probing\":\"ON\"}}"
  Module2 : NCR18650BD_98S45P_Library_lib/Modules/ModuleType1  SOC_vecCell=[0 0.01 0.02 0.03 0.04 0.05 0.06 0.07 0.08 0.09 0.1 0.11 0.12 0.13 0.14 0.15 0.16 0.17 0.18 0.19 0.2 0.21 0.22 0.23 0.24 0.25 0.26 0.27 0.28 0.29 0.3 0.31 0.32 0.33 0.34 0.35 0.36 0.37 0.38 0.39 0.4 0.41 0.42 0.43 0.44 0.45 0.46 0.47 0.48 0.49 0.5 0.51 0.52 0.53 0.54 0.55 0.56 0.57 0.58 0.59 0.6 0.61 0.62 0.63 0.64 0.65 0.66 0.67 0.68 0.69 0.7 0.71 0.72 0.73 0.74 0.75 0.76 0.77 0.78 0.79 0.8 0.81 0.82 0.83 0.84 0.85 0.86 0.87 0.88 0.89 0.9 0.91 0.92 0.93 0.94 0.95 0.96 0.97 0.98 0.99 1]  V0_vecCell=[2.90003 2.94341 2.98679 3.04987 3.09433 3.12791 3.16031 3.20369 3.23862 3.26689 3.29115 3.31383 3.33202 3.35112 3.36833 3.38413 3.39973 3.41137 3.42149 3.43136 3.44073 3.45027 3.46068 3.47113 3.47814 3.48494 3.49199 3.49905 3.50562 3.51187 3.51861 3.52535 3.53209 3.53818 3.54353 3.54849 3.55353 3.55855 3.56357 3.56831 3.57308 3.57787 3.58264 3.58755 3.5925 3.5985 3.60496 3.61149 3.61805 3.6246 3.63116 3.63855 3.64609 3.65336 3.66064 3.66791 3.67613 3.68522 3.69443 3.70367 3.713 3.72241 3.73154 3.74037 3.7492 3.75786 3.76617 3.77556 3.78485 3.79413 3.8034 3.81149 3.81977 3.82804 3.83631 3.84472 3.85317 3.86155 3.86993 3.87831 3.88686 3.89534 3.90461 3.91454 3.92565 3.93721 3.94924 3.96155 3.97383 3.98598 3.99856 4.01117 4.02361 4.03609 4.04694 4.05695 4.06641 4.07551 4.08514 4.09447 4.10453] V  V_rangeCell=[2.25 Inf] V  R0_vecCell=[0.1741 0.15823 0.14313 0.13285 0.12044 0.10641 0.09605 0.09162 0.08758 0.08349 0.08021 0.07738 0.07487 0.07338 0.07189 0.07117 0.0704 0.06898 0.06755 0.06631 0.06509 0.06388 0.06326 0.06281 0.06182 0.06095 0.06025 0.05955 0.05877 0.05807 0.05761 0.05714 0.05668 0.05611 0.05546 0.0549 0.05439 0.05388 0.05337 0.0528 0.05223 0.05165 0.05106 0.05046 0.04986 0.04945 0.04913 0.04883 0.04854 0.04826 0.04797 0.04782 0.04765 0.0473 0.04695 0.04661 0.04638 0.0463 0.04625 0.04621 0.04624 0.04628 0.04628 0.04623 0.04617 0.04599 0.04573 0.0457 0.04568 0.04565 0.04563 0.04535 0.0451 0.04486 0.04461 0.04446 0.04435 0.04423 0.04411 0.044 0.04372 0.04339 0.04323 0.0432 0.04344 0.04374 0.0441 0.04452 0.04494 0.0454 0.04594 0.0463 0.04649 0.04668 0.04629 0.04541 0.04438 0.04326 0.04154 0.03869 0.03326] Ohm  AHCell=3.153 hr*A  extrapolation_optionCell=simscape.enum.extrapolation.nearest  P=45  S=7  iCell_specify=off  iCell_priority=None  iCell=0 A  iCell_nominal_specify=off  iCell_nominal_value=1  iCell_nominal_unit=A  vCell_specify=off  vCell_priority=None  vCell=0 V  vCell_nominal_specify=off  vCell_nominal_value=1  vCell_nominal_unit=V  socCell_specify=off  socCell_priority=High  socCell=1  socCell_nominal_specify=off  socCell_nominal_value=1  socCell_nominal_unit=1  numCyclesCell_specify=off  numCyclesCell_priority=High  numCyclesCell=0  numCyclesCell_nominal_specify=off  numCyclesCell_nominal_value=1  numCyclesCell_nominal_unit=1  vParallelAssembly_specify=off  vParallelAssembly_priority=None  vParallelAssembly=repmat(0, 7, 1) V  vParallelAssembly_nominal_specify=off  vParallelAssembly_nominal_value=1  vParallelAssembly_nominal_unit=V  socParallelAssembly_specify=off  socParallelAssembly_priority=None  socParallelAssembly=repmat(1, 7, 1)  socParallelAssembly_nominal_specify=off  socParallelAssembly_nominal_value=1  socParallelAssembly_nominal_unit=1
      settings: InternalSimscapePortConfiguration="{\"Bottom\":[{\"id\":\"n\",\"label\":\"-\",\"type\":\"foundation.electrical.electrical\"}],\"Left\":[],\"Right\":[],\"Top\":[{\"id\":\"p\",\"label\":\"+\",\"type\":\"foundation.electrical.electrical\"}]}"
  Module2_outputs : SimscapeProbe  BoundBlock=647  Variables="{\"iCell\":{\"Probing\":\"ON\"},\"numCyclesCell\":{\"Probing\":\"ON\"},\"socCell\":{\"Probing\":\"ON\"},\"socParallelAssembly\":{\"Probing\":\"ON\"},\"vCell\":{\"Probing\":\"ON\"},\"vParallelAssembly\":{\"Probing\":\"ON\"}}"
  iCellMux : Mux  Inputs=2
  numCyclesCellMux : Mux  Inputs=2
  socCellMux : Mux  Inputs=2
  socParallelAssemblyMux : Mux  Inputs=2
  vCellMux : Mux  Inputs=2
  vParallelAssemblyMux : Mux  Inputs=2
  + : PMIOPort  Side=Left
  - : PMIOPort  Port=2  Side=Right
  iCell : Outport
  numCyclesCell : Outport  Port=2
  socCell : Outport  Port=3
  socParallelAssembly : Outport  Port=4
  vCell : Outport  Port=5
  vParallelAssembly : Outport  Port=6
  wires:
  Module1_outputs/1 -> [iCell1]
  iCellMux/1 -> iCell/1
  [iCell1] -> iCellMux/1
  Module1_outputs/2 -> [numCyclesCell1]
  numCyclesCellMux/1 -> numCyclesCell/1
  [numCyclesCell1] -> numCyclesCellMux/1
  Module1_outputs/3 -> [socCell1]
  socCellMux/1 -> socCell/1
  [socCell1] -> socCellMux/1
  Module1_outputs/4 -> [socParallelAssembly1]
  socParallelAssemblyMux/1 -> socParallelAssembly/1
  [socParallelAssembly1] -> socParallelAssemblyMux/1
  Module1_outputs/5 -> [vCell1]
  vCellMux/1 -> vCell/1
  [vCell1] -> vCellMux/1
  Module1_outputs/6 -> [vParallelAssembly1]
  vParallelAssemblyMux/1 -> vParallelAssembly/1
  [vParallelAssembly1] -> vParallelAssemblyMux/1
  Module2_outputs/1 -> [iCell2]
  [iCell2] -> iCellMux/2
  Module2_outputs/2 -> [numCyclesCell2]
  [numCyclesCell2] -> numCyclesCellMux/2
  Module2_outputs/3 -> [socCell2]
  [socCell2] -> socCellMux/2
  Module2_outputs/4 -> [socParallelAssembly2]
  [socParallelAssembly2] -> socParallelAssemblyMux/2
  Module2_outputs/5 -> [vCell2]
  [vCell2] -> vCellMux/2
  Module2_outputs/6 -> [vParallelAssembly2]
  [vParallelAssembly2] -> vParallelAssemblyMux/2
  connections:
  Module2/LConn1 -- Module1/RConn1
  Module1/LConn1 -- +/RConn1
  Module2/RConn1 -- -/RConn1
